simulink model "Practica_7simu"  (R2026b)
settings: Solver=VariableStepAuto  StopTime=5
settings Model: LastModifiedBy=JUAN

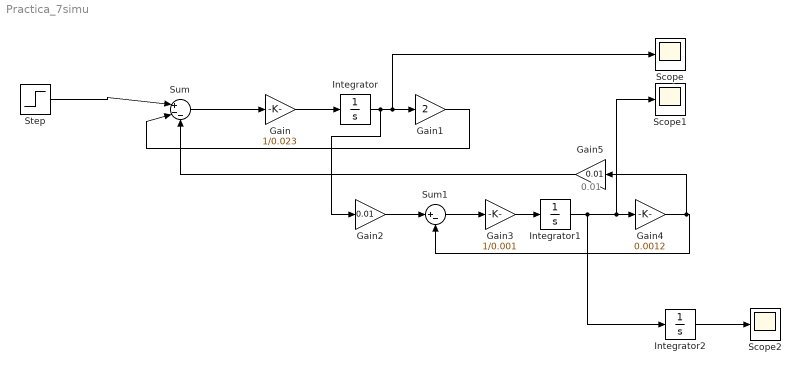
== system Practica_7simu ==
  note: 0.01
  Gain : Gain  Gain=1/0.023
  Gain1 : Gain  Gain=2
  Gain2 : Gain  Gain=0.01
  Gain3 : Gain  Gain=1/0.001
  Gain4 : Gain  Gain=0.0012
  Gain5 : Gain  Gain=0.01
  Integrator : Integrator
  Integrator1 : Integrator
  Integrator2 : Integrator
  Scope : Scope
      settings: ActiveDisplayYMinimum=-0.7499256880532239  ActiveDisplayYMaximum=6.7493311924790165
  Scope1 : Scope
      settings: ActiveDisplayYMinimum=-6.2340073344915918  ActiveDisplayYMaximum=56.106066010424342
  Scope2 : Scope
      settings: ActiveDisplayYMinimum=281.72305927596125  ActiveDisplayYMaximum=544.164479449963  DataLoggingVariableName=ScopeData2
  Step : Step  Time=0  FinalValue=12  SampleTime=0
  Sum : Sum  Inputs=|+--
  Sum1 : Sum  Inputs=|+-
  wires:
  Step/1 -> Sum/1
  Sum/1 -> Gain/1
  Gain/1 -> Integrator/1
  Integrator/1 -> Gain2/1, Scope/1, Gain1/1
  Gain1/1 -> Sum/2
  Gain2/1 -> Sum1/1
  Sum1/1 -> Gain3/1
  Gain3/1 -> Integrator1/1
  Integrator1/1 -> Integrator2/1, Scope1/1, Gain4/1
  Gain4/1 -> Gain5/1, Sum1/2
  Gain5/1 -> Sum/3
  Integrator2/1 -> Scope2/1
